simulink model "variant7_energy_hub"  (R2025b)
settings: Solver=FixedStepDiscrete  StartTime=0.0  StopTime=24  FixedStep=0.25  RelTol=1e-3
model workspace (MAT data in the model file):
  hub_profile = [0 0.25 0.5 0.75 1 1.25 1.5 1.75 2 2.25 2.5 2.75 ... (1164 elements, 97x12)]
settings Model: Creator=zahar  LastModifiedBy=zahar

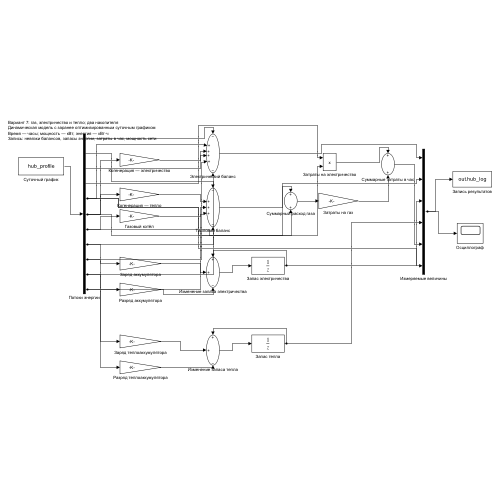
[thumbnail: Simulink's stored preview of the top-level diagram]
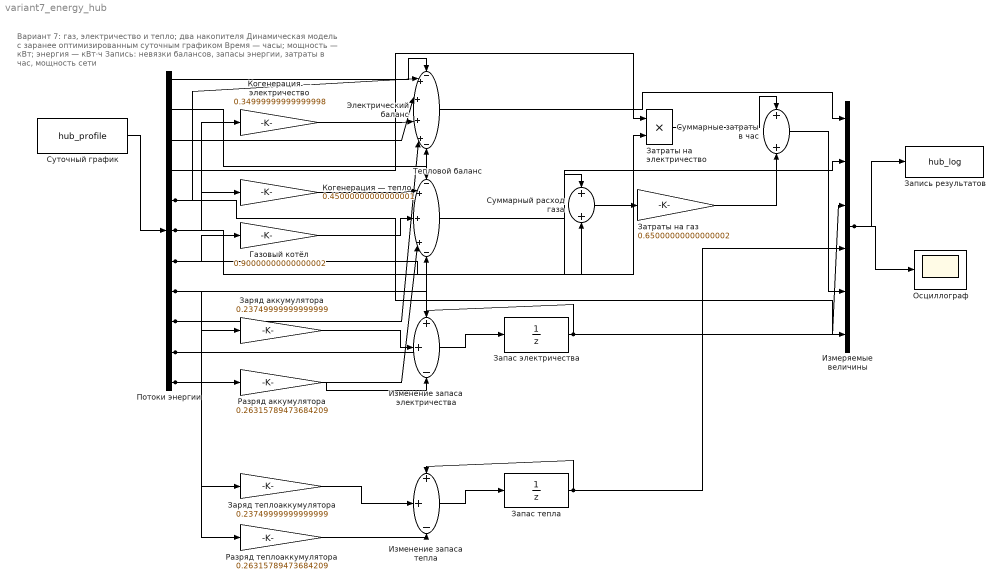
== system variant7_energy_hub ==
  note: Вариант 7: газ, электричество и тепло; два накопителя
      | Динамическая модель с заранее оптимизированным суточным графиком
      | Время — часы; мощность — кВт; энергия — кВт·ч
      | Запись: невязки балансов, запасы энергии, затраты в час, мощность сети
  Газовый котёл : Gain  Gain=0.90000000000000002
  Запас тепла : UnitDelay  SampleTime=0.25  HasFrameUpgradeWarning=on
  Запас электричества : UnitDelay  SampleTime=0.25  HasFrameUpgradeWarning=on
  Запись результатов : ToWorkspace  VariableName=hub_log  SaveFormat=Structure With Time  SampleTime=-1
  Заряд аккумулятора : Gain  Gain=0.23749999999999999
  Заряд теплоаккумулятора : Gain  Gain=0.23749999999999999
  Затраты на газ : Gain  Gain=0.65000000000000002
  Затраты на электричество : Product
  Изменение запаса тепла : Sum  Inputs=++-
  Изменение запаса электричества : Sum  Inputs=++-
  Измеряемые величины : Mux  Inputs=6
  Когенерация — тепло : Gain  Gain=0.45000000000000001
  Когенерация — электричество : Gain  Gain=0.34999999999999998
  Осциллограф : Scope
  Потоки энергии : Demux  Outputs=11
  Разряд аккумулятора : Gain  Gain=0.26315789473684209
  Разряд теплоаккумулятора : Gain  Gain=0.26315789473684209
  Суммарные затраты в час : Sum
  Суммарный расход газа : Sum
  Суточный график : FromWorkspace  VariableName=hub_profile  SampleTime=0.25  Interpolate=off  OutputAfterFinalValue=Holding final value
  Тепловой баланс : Sum  Inputs=-+++-
  Электрический баланс : Sum  Inputs=-++++-
  wires:
  Суточный график/1 -> Потоки энергии/1
  Потоки энергии/6 -> Когенерация — электричество/1, Когенерация — тепло/1, Суммарный расход газа/1
  Потоки энергии/7 -> Газовый котёл/1, Суммарный расход газа/2
  Потоки энергии/1 -> Электрический баланс/1
  Потоки энергии/5 -> Электрический баланс/2, Затраты на электричество/2, Измеряемые величины/6
  Потоки энергии/3 -> Электрический баланс/3
  Когенерация — электричество/1 -> Электрический баланс/4
  Потоки энергии/9 -> Электрический баланс/5, Разряд аккумулятора/1
  Потоки энергии/8 -> Электрический баланс/6, Заряд аккумулятора/1
  Потоки энергии/2 -> Тепловой баланс/1
  Когенерация — тепло/1 -> Тепловой баланс/2
  Газовый котёл/1 -> Тепловой баланс/3
  Потоки энергии/11 -> Тепловой баланс/4, Разряд теплоаккумулятора/1
  Потоки энергии/10 -> Тепловой баланс/5, Заряд теплоаккумулятора/1
  Запас электричества/1 -> Изменение запаса электричества/1, Измеряемые величины/3
  Заряд аккумулятора/1 -> Изменение запаса электричества/2
  Разряд аккумулятора/1 -> Изменение запаса электричества/3
  Изменение запаса электричества/1 -> Запас электричества/1
  Запас тепла/1 -> Изменение запаса тепла/1, Измеряемые величины/4
  Заряд теплоаккумулятора/1 -> Изменение запаса тепла/2
  Разряд теплоаккумулятора/1 -> Изменение запаса тепла/3
  Изменение запаса тепла/1 -> Запас тепла/1
  Потоки энергии/4 -> Затраты на электричество/1
  Суммарный расход газа/1 -> Затраты на газ/1
  Затраты на электричество/1 -> Суммарные затраты в час/1
  Затраты на газ/1 -> Суммарные затраты в час/2
  Электрический баланс/1 -> Измеряемые величины/1
  Тепловой баланс/1 -> Измеряемые величины/2
  Суммарные затраты в час/1 -> Измеряемые величины/5
  Измеряемые величины/1 -> Запись результатов/1, Осциллограф/1
